simulink model "receiver_dsp_testbench"  (R2024b)
settings: Solver=FixedStepDiscrete  StartTime=0.0  StopTime=0.04995  FixedStep=1/20000  RelTol=1e-3
values from neighbouring files (symbols this model uses):
  firCoefficients = fir1(filterOrder, normalizedCutoff, 'low')    [setup_receiver_model.m]
  matchedFilterCoefficients = flip(burst).'    [setup_receiver_model.m]
undefined symbols (not defined in the file or in its folder): dspblkCoreblockFVToolHelper, gcbh
libraries: commchan3 x1, simulink x1
settings Model: Creator=samue  LastModifiedBy=samue

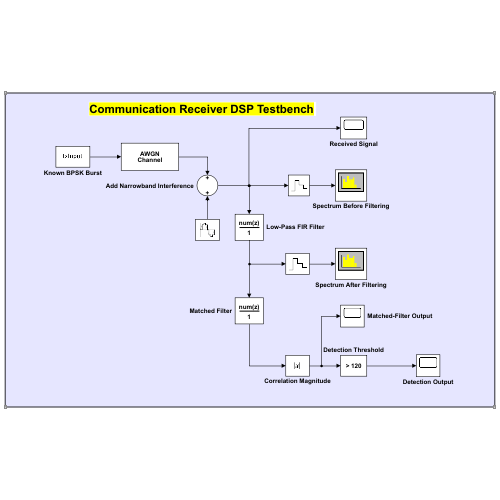
[thumbnail: Simulink's stored preview of the top-level diagram]
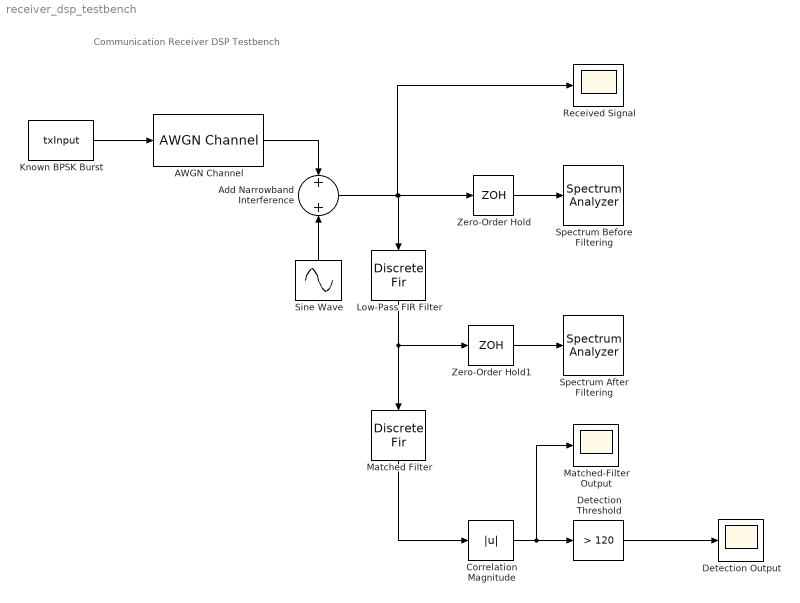
== system receiver_dsp_testbench ==
  note: Communication Receiver DSP Testbench
  AWGN Channel : commchan3/AWGN Channel  LegacyMode=off  NoiseMethod="Signal to noise ratio  (SNR)"  noiseMode="Signal to noise ratio  (SNR)"  EbNo=10  EsNo=10  SNR=10  BitsPerSymbol=1  SignalPower=1  SamplesPerSymbol=1  SymbolPeriod=1  VarianceSource=Parameter  Variance=1  RandomStream=Global stream  Seed=67  SimulateUsing=Interpreted execution
  Add Narrowband Interference : Sum
  Correlation Magnitude : Abs  SaturateOnIntegerOverflow=off
  Detection Output : Scope
  Detection Threshold : simulink/Logic and Bit Operations/Compare To Constant  relop=>  const=120  OutDataTypeStr=boolean
  Known BPSK Burst : FromWorkspace  VariableName=txInput  Interpolate=off  OutputAfterFinalValue=Holding final value
  Low-Pass FIR Filter : DiscreteFir  LoadFcn=dspblkCoreblockFVToolHelper(gcbh,'load');  Coefficients=firCoefficients
      settings: CopyFcn=dspblkCoreblockFVToolHelper(gcbh,'copy');  DeleteFcn=dspblkCoreblockFVToolHelper(gcbh,'close');  ModelCloseFcn=dspblkCoreblockFVToolHelper(gcbh,'close');  PreSaveFcn=dspblkCoreblockFVToolHelper(gcbh,'presave');  PostSaveFcn=dspblkCoreblockFVToolHelper(gcbh,'postsave');  CloseFcn=dspblkCoreblockFVToolHelper(gcbh,'close');
  Matched Filter : DiscreteFir  LoadFcn=dspblkCoreblockFVToolHelper(gcbh,'load');  Coefficients=matchedFilterCoefficients
      settings: CopyFcn=dspblkCoreblockFVToolHelper(gcbh,'copy');  DeleteFcn=dspblkCoreblockFVToolHelper(gcbh,'close');  ModelCloseFcn=dspblkCoreblockFVToolHelper(gcbh,'close');  PreSaveFcn=dspblkCoreblockFVToolHelper(gcbh,'presave');  PostSaveFcn=dspblkCoreblockFVToolHelper(gcbh,'postsave');  CloseFcn=dspblkCoreblockFVToolHelper(gcbh,'close');
  Matched-Filter Output : Scope
  Received Signal : Scope
  Sine Wave : Sin  Amplitude=0.8  Frequency=2*pi*4000  SampleTime=1/20000
  Spectrum After Filtering : SpectrumAnalyzer  WindowPosition=[517.000000,302.000000,800.000000,500.000000,]  ScopeFrameLocation=window  PlotAsTwoSidedSpectrum=off  WindowInvariantSamplesPerUpdate=on  CenterFrequency=5000  StartFrequency=0  StopFrequency=10000  YLimits=[-62.07846333,20.63539175]  SelectedToolstripTab=spectrumAnalyzerToolstrip.measurementsTab
  Spectrum Before Filtering : SpectrumAnalyzer  WindowPosition=[9.000000,225.000000,849.000000,448.000000,]  ScopeFrameLocation=window  PlotAsTwoSidedSpectrum=off  WindowInvariantSamplesPerUpdate=on  CenterFrequency=5000  StartFrequency=0  StopFrequency=10000  YLimits=[-38.757041,31.55205667]  SelectedToolstripTab=spectrumAnalyzerToolstrip.spectrumTab
  Zero-Order Hold : ZeroOrderHold  SampleTime=1/20000
  Zero-Order Hold1 : ZeroOrderHold  SampleTime=1/20000
  wires:
  Known BPSK Burst/1 -> AWGN Channel/1
  AWGN Channel/1 -> Add Narrowband Interference/1
  Sine Wave/1 -> Add Narrowband Interference/2
  Zero-Order Hold/1 -> Spectrum Before Filtering/1
  Low-Pass FIR Filter/1 -> Matched Filter/1, Zero-Order Hold1/1
  Zero-Order Hold1/1 -> Spectrum After Filtering/1
  Matched Filter/1 -> Correlation Magnitude/1
  Correlation Magnitude/1 -> Matched-Filter Output/1, Detection Threshold/1
  Detection Threshold/1 -> Detection Output/1
  Add Narrowband Interference/1 -> Received Signal/1, Zero-Order Hold/1, Low-Pass FIR Filter/1
